simulink model "boost_openloop"  (R2025a)
settings: Solver=FixedStepAuto  StartTime=0.0  StopTime=T_sim  FixedStep=Ts_pwr  RelTol=1e-3
values from neighbouring files (symbols this model uses):
  C = 220e-6    (= 0.00022)    [param_boost_pblb.m]
  D_nom = 1 - Vin_nom/Vref    (= 0.5)    [param_boost_pblb.m]
  L = 680e-6    (= 0.00068)    [param_boost_pblb.m]
  R_nom = 32    [param_boost_pblb.m]    (also in uji_skenario.m)
  Ts_pwr = 5e-7    (= 5e-07)    [param_boost_pblb.m]    (also in tuning_pid.m; uji_skenario.m = 2e-07)
  Vin_nom = 24    [param_boost_pblb.m]    (also in uji_skenario.m)
libraries: spsSeriesRLCBranchLib x3, spsGroundLib x2, spsCurrentMeasurementLib x2, spsDCVoltageSourceLib x1, spsDiodeLib x1, spsMosfetLib x1, spsPWMGeneratorDCDCLib x1, spsVoltageMeasurementLib x1, sps_lib x1
settings Model: Creator=first  LastModifiedBy=first
settings DataIOCC: SignalLogging=off

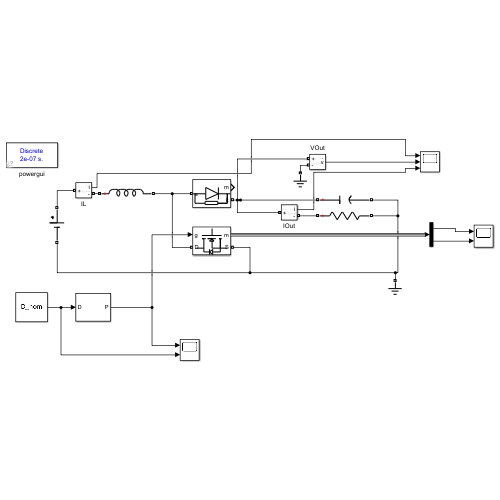
[thumbnail: Simulink's stored preview of the top-level diagram]
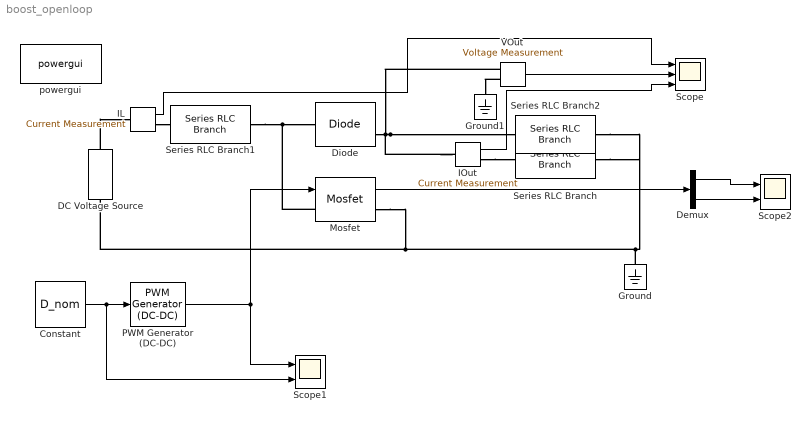
== system boost_openloop ==
  Constant : Constant  Value=D_nom
  DC Voltage Source : spsDCVoltageSourceLib/DC Voltage Source  Amplitude=Vin_nom  Measurements=None
  Demux : Demux  Outputs=2
  Diode : spsDiodeLib/Diode  Ron=Ron_D  Lon=0  Vf=Vf_D  IC=0  UseSnubber=0  Rs=1e5  Cs=inf  Measurements=on
  Ground : spsGroundLib/Ground  LConnTagsString=a
  Ground1 : spsGroundLib/Ground  LConnTagsString=a
  IL : spsCurrentMeasurementLib/Current Measurement  PhasorSimulation=off  OutputType=Complex  PSBequivalent=0
  IOut : spsCurrentMeasurementLib/Current Measurement  PhasorSimulation=off  OutputType=Complex  PSBequivalent=0
  Mosfet : spsMosfetLib/Mosfet  Ron=Ron_Q  Lon=0  Rd=0.01  Vfd=0  IC=0  Rs=1e5  Cs=inf  Measurements=on
  PWM Generator (DC-DC) : spsPWMGeneratorDCDCLib/PWM Generator (DC-DC)  Fsw=fsw  Ts=0
  Scope : Scope  NumInputPorts=3
      settings: ActiveDisplayYMinimum=-1  ActiveDisplayYMaximum=1  DataLoggingDecimation=10
  Scope1 : Scope  NumInputPorts=2
      settings: ActiveDisplayYMinimum=0  ActiveDisplayYMaximum=1.3  DataLoggingDecimation=10
  Scope2 : Scope  NumInputPorts=2
      settings: ActiveDisplayYMinimum=-1.950111165493172  ActiveDisplayYMaximum=17.548401674148955  DataLoggingDecimation=10  DataLoggingVariableName=ScopeData2
  Series RLC Branch : spsSeriesRLCBranchLib/Series RLC Branch  LConnTagsString=__new0  RConnTagsString=__new0  BranchType=R  Resistance=R_nom  Inductance=1e-3  SetiL0=off  InitialCurrent=0  Capacitance=1e-6  Setx0=off  InitialVoltage=0  Measurements=None
  Series RLC Branch1 : spsSeriesRLCBranchLib/Series RLC Branch  LConnTagsString=__new0  RConnTagsString=__new0  BranchType=L  Resistance=1  Inductance=L  SetiL0=off  InitialCurrent=0  Capacitance=1e-6  Setx0=off  InitialVoltage=0  Measurements=None
  Series RLC Branch2 : spsSeriesRLCBranchLib/Series RLC Branch  LConnTagsString=__new0  RConnTagsString=__new0  BranchType=C  Resistance=1  Inductance=1e-3  SetiL0=off  InitialCurrent=0  Capacitance=C  Setx0=on  InitialVoltage=Vc0  Measurements=None
  VOut : spsVoltageMeasurementLib/Voltage Measurement  PhasorSimulation=off  OutputType=Complex  PSBequivalent=0
  powergui : sps_lib/powergui  Priority=1  SimulationMode=Discrete  SampleTime=Ts_pwr  frequency=60  Iterations=50  frequencyindice=0  Pbase=100e6  ErrMax=1e-4  UnitsV=kV  UnitsW=MW  buscounter=0  FunctionMessages=off  echomessages=off  EnableUseOfTLC=off  CurrentSourceSwitches=off  DisableSnubberDevices=off  DisableRonSwitches=off  DisableVfSwitches=off  DisplayEquations=off  AutomaticDiscreteSolvers=off  SolverType=Tustin/Backward Euler (TBE)  Interpol=off  ExternalGateDelay=off  methode=off  Ts=100  x0status=blocks  SPID=on  SwTol=0  HookPort=off  NonlinearTolerance=1e-4  nMaxIteration=100  ContinueOnMaxIteration=off  RestoreLinks=warning  ResistiveCurrentMeasurement=off  Frange=[0:2:500]  Ylog=off  Xlog=on  ShowGrid=off  save=off  variable=ZData  structure=0  ZoomFFT=off  StartTime=0.0  cycles=1  DisplayStyle=1  fundamental=60  FreqAxis=off  MaxFrequency=1000  frequencyindicesteady=1  RmsSteady=1  display=off
  wires:
  Constant/1 -> Scope1/2, PWM Generator (DC-DC)/1
  PWM Generator (DC-DC)/1 -> Mosfet/1, Scope1/1
  VOut/1 -> Scope/2
  IOut/1 -> Scope/3
  IL/1 -> Scope/1
  Demux/1 -> Scope2/1
  Demux/2 -> Scope2/2
  Mosfet/1 -> Demux/1
  connections:
  Series RLC Branch1/RConn1 -- Mosfet/LConn1 -- Diode/LConn1
  Diode/RConn1 -- Series RLC Branch2/LConn1 -- IOut/LConn1 -- VOut/LConn1
  Ground/LConn1 -- Mosfet/RConn1 -- DC Voltage Source/LConn1 -- Series RLC Branch/RConn1 -- Series RLC Branch2/RConn1
  VOut/LConn2 -- Ground1/LConn1
  IL/RConn1 -- Series RLC Branch1/LConn1
  DC Voltage Source/RConn1 -- IL/LConn1
  IOut/RConn1 -- Series RLC Branch/LConn1
